simulink model "power_shuffler_sim"  (R2025b)
settings: Solver=VariableStepAuto  StartTime=0.0  StopTime=0.15  MaxStep=1e-4  RelTol=1e-4
PreLoadFcn:
  | P = init_params; CTRL_MODE = 1;
libraries: fl_lib x74, ee_lib x53, nesl_utility x50
(part 1 of 6)
settings Model: SimulationMode=accelerator  Creator=jazsa  LastModifiedBy=jazsa
settings SolverCC: ZeroCrossAlgorithm=Adaptive
settings DataIOCC: SignalLogging=off

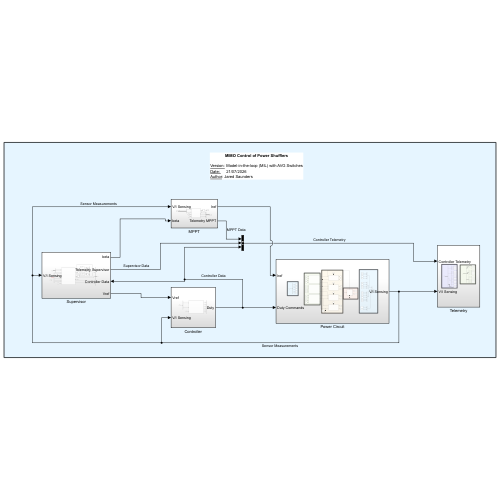
[thumbnail: Simulink's stored preview of the top-level diagram]
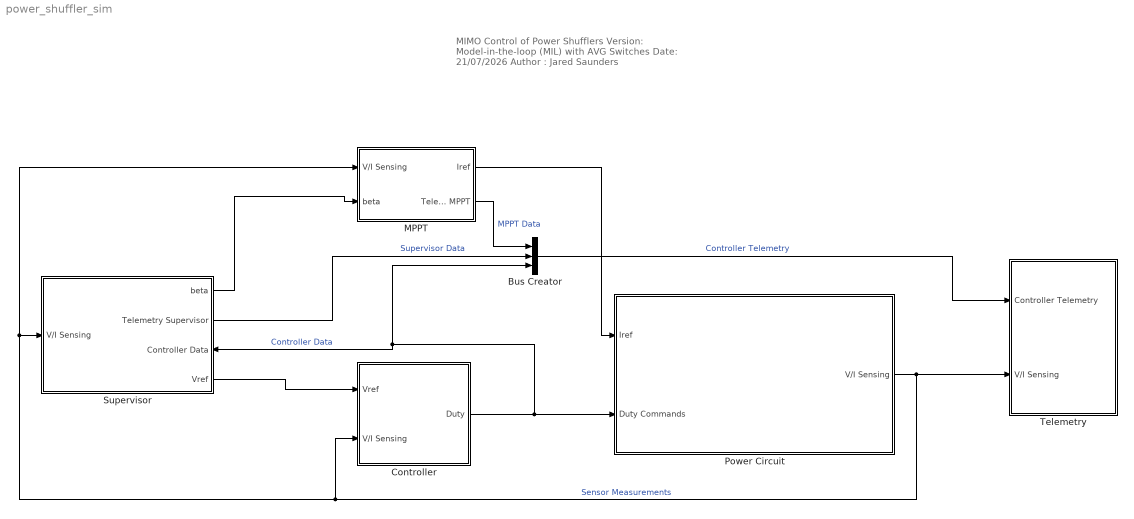
== system power_shuffler_sim ==
  note: MIMO Control of Power Shufflers
      |
      | Version: Model-in-the-loop (MIL) with AVG Switches
      | Date: 21/07/2026
      | Author : Jared Saunders
  Bus Creator : BusCreator  Inputs=3
  Controller : Subsystem
  MPPT : Subsystem
  Power Circuit : Subsystem
  Supervisor : Subsystem
      settings: PortSchema="{\"entries\":[{\"content\":{\"sides\":[{\"content\":{\"connectorIds\":[\"In1\"]},\"type\":\"ConnectorPlacement.EquallySpacedRectSide\",\"uuid\":\"4149ece3-2139-4a6b-be3b-85e3b5016338\"},{\"content\":{\"connectorIds\":[\"Out1\",\"Out2\",\"In2\",\"Out3\"],\"side\":\"RIGHT\"},\"type\":\"ConnectorPlacement.EquallySpacedRectSide\",\"uuid\":\"a4c8f16e-63c5-4e73-b921-9be0544bd052\"},{\"content\":{\"side\":\"TOP\"},\"type\":\"ConnectorPlacement.EquallySpacedRectSide\",\"uuid\":\"efcb0ad6-b028-42ed-a2aa-71b179d48e39\"}]},\"type\":\"ConnectorPlacement.EquallySpacedConnector\",\"uuid\":\"3400d1fe-81e3-4212-a4bc-db484173b6e0\"}],\"packageUris\":[\"http://schema.mathworks.com/mf0/Connector/R2020b\"],\"version\":\"1.0\"}"
  Telemetry : Subsystem
  wires:
  MPPT/1(Iref) -> Power Circuit/1(Iref)
  Supervisor/1(beta) -> MPPT/2(beta)
  Power Circuit/1(V/I Sensing) -> Telemetry/2(V/I Sensing), Controller/2(V/I Sensing), MPPT/1(V/I Sensing), Supervisor/1(V/I Sensing)  "Sensor Measurements"
  Supervisor/3(Vref) -> Controller/1(Vref)
  Controller/1(Duty) -> Power Circuit/2(Duty Commands), Bus Creator/3, Supervisor/2(Controller Data)  "Controller Data"
  MPPT/2(Telemetry MPPT) -> Bus Creator/1  "MPPT Data"
  Supervisor/2(Telemetry Supervisor) -> Bus Creator/2  "Supervisor Data"
  Bus Creator/1 -> Telemetry/1(Controller Telemetry)  "Controller Telemetry"

== system power_shuffler_sim/Controller ==
  Vref : Inport
  V/I Sensing : Inport  Port=2
  Bus Creator : BusCreator  Inputs=6
  Bus Selector : BusSelector  OutputSignals=Module Voltages,Phase Currents
  Controller : MATLAB Function  TreatAsAtomicUnit=on  SystemSampleTime=50e-6
  Duty : Outport
  wires:
  Bus Selector/1 -> Controller/1(VM)  "<Module Voltages>"
  Controller/6(dB3) -> Bus Creator/6
  Controller/5(dA3) -> Bus Creator/5
  Controller/4(dB2) -> Bus Creator/4
  Controller/3(dA2) -> Bus Creator/3
  Controller/2(dB1) -> Bus Creator/2
  Controller/1(dA1) -> Bus Creator/1
  Bus Creator/1 -> Duty/1
  V/I Sensing/1 -> Bus Selector/1
  Bus Selector/2 -> Controller/2(IL)  "<Phase Currents>"
  Vref/1 -> Controller/3(rv)

== system power_shuffler_sim/MPPT ==
  V/I Sensing : Inport
  beta : Inport  Port=2
  Bus Creator : BusCreator  Inputs=3
  Bus Selector : BusSelector  OutputSignals=String Power Meter
  Bus Selector1 : BusSelector  OutputSignals=V_string,I_string
  Delay : UnitDelay  InitialCondition=12  SampleTime=1e-3  HasFrameUpgradeWarning=on
  Enable : Constant
  P&O : MATLAB Function  TreatAsAtomicUnit=on  SystemSampleTime=1e-3
  Iref : Outport
  Telemetry MPPT : Outport  Port=2
  wires:
  beta/1 -> P&O/3(beta)
  V/I Sensing/1 -> Bus Selector/1
  P&O/3(state) -> Bus Creator/3
  Bus Selector1/1 -> P&O/1(Vstr)  "<V_string>"
  Bus Selector1/2 -> P&O/2(Istr)  "<I_string>"
  P&O/1(Iref) -> Bus Creator/1, Delay/1
  Delay/1 -> Iref/1
  Enable/1 -> P&O/4(en)
  Bus Creator/1 -> Telemetry MPPT/1
  P&O/2(Pav) -> Bus Creator/2
  Bus Selector/1 -> Bus Selector1/1  "<String Power Meter>"

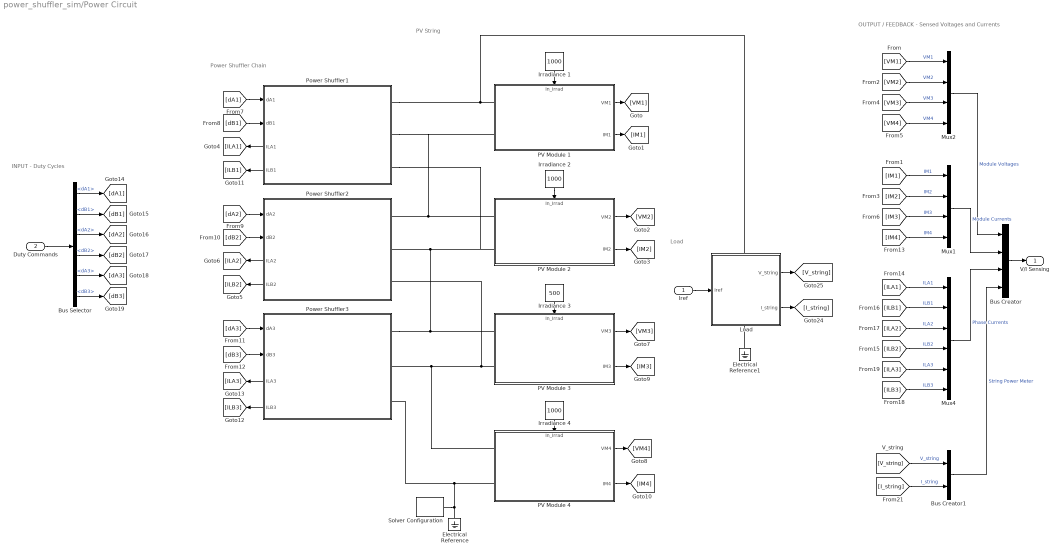
== system power_shuffler_sim/Power Circuit ==
  note: OUTPUT / FEEDBACK - Sensed Voltages and Currents
  note: Load
  note: PV String
  note: Power Shuffler Chain
  note: INPUT - Duty Cycles
  Iref : Inport
  Duty Commands : Inport  Port=2
  Bus Creator : BusCreator  Inputs=4
  Bus Creator1 : BusCreator  Inputs=2
  Bus Selector : BusSelector  OutputSignals=dA1,dB1,dA2,dB2,dA3,dB3
  Electrical Reference : fl_lib/Electrical/Electrical Elements/Electrical Reference
  Electrical Reference1 : fl_lib/Electrical/Electrical Elements/Electrical Reference
  Irradiance 1 : Constant  Value=1000
  Irradiance 2 : Constant  Value=1000
  Irradiance 3 : Constant  Value=500
  Irradiance 4 : Constant  Value=1000
  Load : Subsystem
      settings: PortSchema="{\"entries\":[{\"content\":{\"sides\":[{\"content\":{\"connectorIds\":[\"LConn1\"]},\"type\":\"ConnectorPlacement.EquallySpacedRectSide\",\"uuid\":\"6f5f716f-38b7-43f9-a9ba-568c6ccf5920\"},{\"content\":{\"connectorIds\":[\"RConn1\"],\"side\":\"RIGHT\"},\"type\":\"ConnectorPlacement.EquallySpacedRectSide\",\"uuid\":\"74a237b1-90a9-413f-978d-7052f4ba1489\"},{\"content\":{\"connectorIds\":[\"In1\"],\"side\":\"TOP\"},\"type\":\"ConnectorPlacement.EquallySpacedRectSide\",\"uuid\":\"e5fcb88f-496e-42e0-91fa-e640406c50d5\"},{\"content\":{\"connectorIds\":[\"Out1\",\"Out2\"],\"side\":\"BOTTOM\"},\"type\":\"ConnectorPlacement.EquallySpacedRectSide\",\"uuid\":\"aed6b45d-7ab9-4ae0-b4e0-d20dd58bb9bf\"}]},\"type\":\"ConnectorPlacement.EquallySpacedConnector\",\"uuid\":\"f6ffe9ce-5007-4054-8c52-fa2588b4e46b\"}],\"packageUris\":[\"http://schema.mathworks.com/mf0/Connector/R2020b\"],\"version\":\"1.0\"}"
  Mux1 : Mux
  Mux2 : Mux
  Mux4 : Mux  Inputs=6
  PV Module 1 : Subsystem
      settings: PortSchema="{\"entries\":[{\"content\":{\"sides\":[{\"content\":{\"connectorIds\":[\"LConn1\",\"LConn2\"]},\"type\":\"ConnectorPlacement.EquallySpacedRectSide\",\"uuid\":\"00bc81be-eb87-4e0d-8cf1-aaf392b111b3\"},{\"content\":{\"connectorIds\":[\"Out1\",\"Out2\"],\"side\":\"RIGHT\"},\"type\":\"ConnectorPlacement.EquallySpacedRectSide\",\"uuid\":\"136cfb59-61d1-4be5-a5a1-62fe670dfe2d\"},{\"content\":{\"connectorIds\":[\"In1\"],\"side\":\"TOP\"},\"type\":\"ConnectorPlacement.EquallySpacedRectSide\",\"uuid\":\"1fa490a3-fddf-446b-98a1-153f2ac018d8\"}]},\"type\":\"ConnectorPlacement.EquallySpacedConnector\",\"uuid\":\"e6ea07bf-3162-47e8-af67-1b2f68d57f24\"}],\"packageUris\":[\"http://schema.mathworks.com/mf0/Connector/R2020b\"],\"version\":\"1.0\"}"
  PV Module 2 : Subsystem
      settings: PortSchema="{\"entries\":[{\"content\":{\"sides\":[{\"content\":{\"connectorIds\":[\"LConn1\",\"LConn2\"]},\"type\":\"ConnectorPlacement.EquallySpacedRectSide\",\"uuid\":\"00bc81be-eb87-4e0d-8cf1-aaf392b111b3\"},{\"content\":{\"connectorIds\":[\"Out1\",\"Out2\"],\"side\":\"RIGHT\"},\"type\":\"ConnectorPlacement.EquallySpacedRectSide\",\"uuid\":\"136cfb59-61d1-4be5-a5a1-62fe670dfe2d\"},{\"content\":{\"connectorIds\":[\"In1\"],\"side\":\"TOP\"},\"type\":\"ConnectorPlacement.EquallySpacedRectSide\",\"uuid\":\"1fa490a3-fddf-446b-98a1-153f2ac018d8\"}]},\"type\":\"ConnectorPlacement.EquallySpacedConnector\",\"uuid\":\"e6ea07bf-3162-47e8-af67-1b2f68d57f24\"}],\"packageUris\":[\"http://schema.mathworks.com/mf0/Connector/R2020b\"],\"version\":\"1.0\"}"
  PV Module 3 : Subsystem
      settings: PortSchema="{\"entries\":[{\"content\":{\"sides\":[{\"content\":{\"connectorIds\":[\"LConn1\",\"LConn2\"]},\"type\":\"ConnectorPlacement.EquallySpacedRectSide\",\"uuid\":\"00bc81be-eb87-4e0d-8cf1-aaf392b111b3\"},{\"content\":{\"connectorIds\":[\"Out1\",\"Out2\"],\"side\":\"RIGHT\"},\"type\":\"ConnectorPlacement.EquallySpacedRectSide\",\"uuid\":\"136cfb59-61d1-4be5-a5a1-62fe670dfe2d\"},{\"content\":{\"connectorIds\":[\"In1\"],\"side\":\"TOP\"},\"type\":\"ConnectorPlacement.EquallySpacedRectSide\",\"uuid\":\"1fa490a3-fddf-446b-98a1-153f2ac018d8\"}]},\"type\":\"ConnectorPlacement.EquallySpacedConnector\",\"uuid\":\"e6ea07bf-3162-47e8-af67-1b2f68d57f24\"}],\"packageUris\":[\"http://schema.mathworks.com/mf0/Connector/R2020b\"],\"version\":\"1.0\"}"
  PV Module 4 : Subsystem
      settings: PortSchema="{\"entries\":[{\"content\":{\"sides\":[{\"content\":{\"connectorIds\":[\"LConn1\",\"LConn2\"]},\"type\":\"ConnectorPlacement.EquallySpacedRectSide\",\"uuid\":\"00bc81be-eb87-4e0d-8cf1-aaf392b111b3\"},{\"content\":{\"connectorIds\":[\"Out1\",\"Out2\"],\"side\":\"RIGHT\"},\"type\":\"ConnectorPlacement.EquallySpacedRectSide\",\"uuid\":\"136cfb59-61d1-4be5-a5a1-62fe670dfe2d\"},{\"content\":{\"connectorIds\":[\"In1\"],\"side\":\"TOP\"},\"type\":\"ConnectorPlacement.EquallySpacedRectSide\",\"uuid\":\"1fa490a3-fddf-446b-98a1-153f2ac018d8\"}]},\"type\":\"ConnectorPlacement.EquallySpacedConnector\",\"uuid\":\"e6ea07bf-3162-47e8-af67-1b2f68d57f24\"}],\"packageUris\":[\"http://schema.mathworks.com/mf0/Connector/R2020b\"],\"version\":\"1.0\"}"
  Power Shuffler1 : Subsystem
      settings: PortSchema="{\"entries\":[{\"content\":{\"sides\":[{\"content\":{\"connectorIds\":[\"LConn1\",\"LConn2\",\"LConn3\"]},\"type\":\"ConnectorPlacement.EquallySpacedRectSide\",\"uuid\":\"00177d11-8382-42fd-b27c-fc09158175e4\"},{\"content\":{\"connectorIds\":[\"In1\",\"In2\",\"Out1\",\"Out2\"],\"side\":\"RIGHT\"},\"type\":\"ConnectorPlacement.EquallySpacedRectSide\",\"uuid\":\"90a306f0-da10-41e1-a725-cfb753adc00c\"},{\"content\":{\"side\":\"TOP\"},\"type\":\"ConnectorPlacement.EquallySpacedRectSide\",\"uuid\":\"612e5683-3ee7-4398-9a5a-0cbdc6c6e41b\"}]},\"type\":\"ConnectorPlacement.EquallySpacedConnector\",\"uuid\":\"1790a0ac-9047-4198-9955-1e7cd181ed81\"}],\"packageUris\":[\"http://schema.mathworks.com/mf0/Connector/R2020b\"],\"version\":\"1.0\"}"
  Power Shuffler2 : Subsystem
      settings: PortSchema="{\"entries\":[{\"content\":{\"sides\":[{\"content\":{\"connectorIds\":[\"LConn1\",\"LConn2\",\"LConn3\"]},\"type\":\"ConnectorPlacement.EquallySpacedRectSide\",\"uuid\":\"00177d11-8382-42fd-b27c-fc09158175e4\"},{\"content\":{\"connectorIds\":[\"In1\",\"In2\",\"Out1\",\"Out2\"],\"side\":\"RIGHT\"},\"type\":\"ConnectorPlacement.EquallySpacedRectSide\",\"uuid\":\"90a306f0-da10-41e1-a725-cfb753adc00c\"},{\"content\":{\"side\":\"TOP\"},\"type\":\"ConnectorPlacement.EquallySpacedRectSide\",\"uuid\":\"612e5683-3ee7-4398-9a5a-0cbdc6c6e41b\"}]},\"type\":\"ConnectorPlacement.EquallySpacedConnector\",\"uuid\":\"1790a0ac-9047-4198-9955-1e7cd181ed81\"}],\"packageUris\":[\"http://schema.mathworks.com/mf0/Connector/R2020b\"],\"version\":\"1.0\"}"
  Power Shuffler3 : Subsystem
      settings: PortSchema="{\"entries\":[{\"content\":{\"sides\":[{\"content\":{\"connectorIds\":[\"LConn1\",\"LConn2\",\"LConn3\"]},\"type\":\"ConnectorPlacement.EquallySpacedRectSide\",\"uuid\":\"00177d11-8382-42fd-b27c-fc09158175e4\"},{\"content\":{\"connectorIds\":[\"In1\",\"In2\",\"Out1\",\"Out2\"],\"side\":\"RIGHT\"},\"type\":\"ConnectorPlacement.EquallySpacedRectSide\",\"uuid\":\"90a306f0-da10-41e1-a725-cfb753adc00c\"},{\"content\":{\"side\":\"TOP\"},\"type\":\"ConnectorPlacement.EquallySpacedRectSide\",\"uuid\":\"612e5683-3ee7-4398-9a5a-0cbdc6c6e41b\"}]},\"type\":\"ConnectorPlacement.EquallySpacedConnector\",\"uuid\":\"1790a0ac-9047-4198-9955-1e7cd181ed81\"}],\"packageUris\":[\"http://schema.mathworks.com/mf0/Connector/R2020b\"],\"version\":\"1.0\"}"
  Solver Configuration : nesl_utility/Solver Configuration  PhysicalDomain=network_engine_domain  SubClassName=solver  LeftPortType=input  RightPortType=generic  Tones=[]  Harmonics=[]  SimulateNoise=off  Profile=off  UseLocalSampling=off  EnableSwitchedLinearOptims=on  FrequencyDomain=off  UseCCode=off  RelTol=0.001  AbsTol=0.001  MinStep=1e-09  ToWorkspace=off  RevertToSquareIcSolve=off  NumHomotopyIterations=100  PhasorMode=off  PhasorModeNumHarmonics=1  ConsistencySolver=NEWTON_XTOL_AFTER_FTOL  IndexReductionMethod=DerivativeReplacement  DoDC=off  ResidualTolerance=1e-09  ConsistencyTolSource=GLOBAL  ConsistencyAbsTol=0.001  ConsistencyRelTol=0.001  ConsistencyTolFactor=0.001  UseLocalSolver=on  LocalSolverChoice=NE_BACKWARD_EULER_ADVANCER  ResolveIndetEquations=on  FunctionEvalNumThread=1  LocalSolverSampleTime=1e-7  DoFixedCost=off  MaxNonlinIter=3  MaxModeIter=2  ComputeImpulses=off  ImpulseIterations=2  LinearAlgebra=auto  LinearAlgebraNumThread=0  EquationFormulation=NE_TIME_EF  DelaysMemoryBudget=1024  AutomaticFiltering=on  FilteringTimeConstant=0.001  PartitionStorageMethod=AS_NEEDED  PartitionMemoryBudget=1024  PartitionMethod=ROBUST  MultibodyUseLocalSolver=off  MultibodyLocalSolverChoice=ODE1  MultibodyLocalSolverSampleTime=0.001
  V/I Sensing : Outport
  wires:
  Iref/1 -> Load/1(Iref)
  Load/2(V_String) -> [V_string]
  PV Module 1/1(VM1) -> [VM1]
  Load/1(I_string) -> [I_string]
  Irradiance 3/1 -> PV Module 3/1(In_Irrad)
  Irradiance 4/1 -> PV Module 4/1(In_Irrad)
  Irradiance 2/1 -> PV Module 2/1(In_Irrad)
  Irradiance 1/1 -> PV Module 1/1(In_Irrad)
  Mux2/1 -> Bus Creator/1  "Module Voltages"
  Mux1/1 -> Bus Creator/2  "Module Currents"
  [VM1] -> Mux2/1  "VM1"
  PV Module 1/2(IM1) -> [IM1]
  [IM1] -> Mux1/1  "IM1"
  PV Module 2/1(VM2) -> [VM2]
  [VM2] -> Mux2/2  "VM2"
  PV Module 2/2(IM2) -> [IM2]
  [VM3] -> Mux2/3  "VM3"
  [IM2] -> Mux1/2  "IM2"
  PV Module 3/1(VM3) -> [VM3]
  PV Module 4/1(VM4) -> [VM4]
  [VM4] -> Mux2/4  "VM4"
  PV Module 3/2(IM3) -> [IM3]
  [IM3] -> Mux1/3  "IM3"
  PV Module 4/2(IM4) -> [IM4]
  [IM4] -> Mux1/4  "IM4"
  Power Shuffler1/1(ILA1) -> [ILA1]
  Power Shuffler1/2(ILB1) -> [ILB1]
  Power Shuffler2/2(ILB2) -> [ILB2]
  Power Shuffler2/1(ILA2) -> [ILA2]
  Power Shuffler3/2(ILB3) -> [ILB3]
  Power Shuffler3/1(ILA3) -> [ILA3]
  [ILB3] -> Mux4/6  "ILB3"
  [ILA3] -> Mux4/5  "ILA3"
  [ILA1] -> Mux4/1  "ILA1"
  [ILA2] -> Mux4/3  "ILA2"
  [ILB1] -> Mux4/2  "ILB1"
  [ILB2] -> Mux4/4  "ILB2"
  Mux4/1 -> Bus Creator/3  "Phase Currents"
  [dA1] -> Power Shuffler1/1(dA1)
  Duty Commands/1 -> Bus Selector/1
  Bus Selector/1 -> [dA1]  "<dA1>"
  Bus Selector/2 -> [dB1]  "<dB1>"
  [dB1] -> Power Shuffler1/2(dB1)
  [dB2] -> Power Shuffler2/2(dB2)
  [dA2] -> Power Shuffler2/1(dA2)
  [dA3] -> Power Shuffler3/1(dA3)
  [dB3] -> Power Shuffler3/2(dB3)
  Bus Selector/4 -> [dB2]  "<dB2>"
  Bus Selector/3 -> [dA2]  "<dA2>"
  Bus Selector/6 -> [dB3]  "<dB3>"
  Bus Selector/5 -> [dA3]  "<dA3>"
  [V_string] -> Bus Creator1/1  "V_string"
  [I_string] -> Bus Creator1/2  "I_string"
  Bus Creator/1 -> V/I Sensing/1
  Bus Creator1/1 -> Bus Creator/4  "String Power Meter"
  connections:
  PV Module 1/LConn2 -- Power Shuffler1/LConn2 -- PV Module 2/LConn1 -- Power Shuffler2/LConn1
  PV Module 1/LConn1 -- Load/RConn1 -- Power Shuffler1/LConn1
  PV Module 3/LConn1 -- PV Module 2/LConn2 -- Power Shuffler1/LConn3 -- Power Shuffler2/LConn2 -- Power Shuffler3/LConn1
  Solver Configuration/RConn1 -- Power Shuffler3/LConn3 -- PV Module 4/LConn2 -- Electrical Reference/LConn1
  PV Module 3/LConn2 -- PV Module 4/LConn1 -- Power Shuffler3/LConn2 -- Power Shuffler2/LConn3
  Electrical Reference1/LConn1 -- Load/LConn1

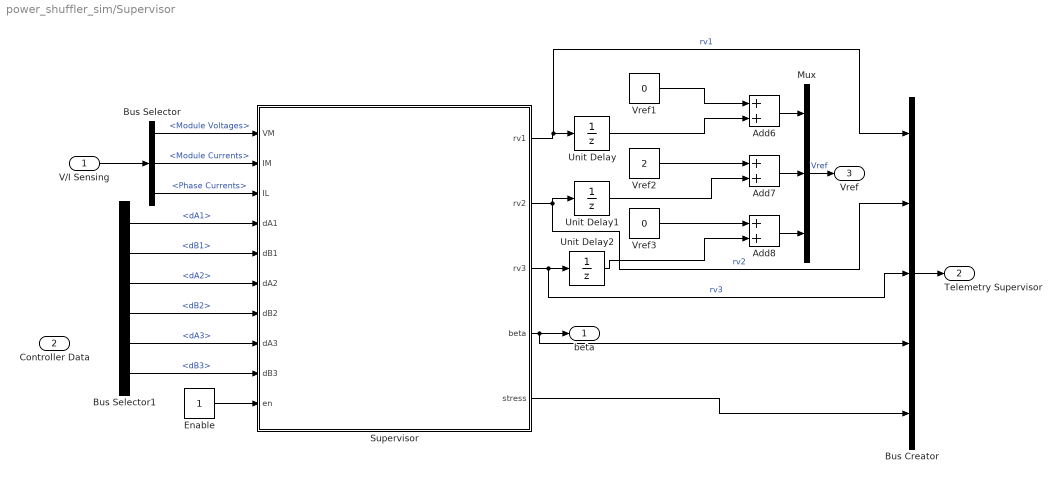
== system power_shuffler_sim/Supervisor ==
  V/I Sensing : Inport
  Controller Data : Inport  Port=2
  Add6 : Sum
  Add7 : Sum
  Add8 : Sum
  Bus Creator : BusCreator  Inputs=5
  Bus Selector : BusSelector  OutputSignals=Module Voltages,Module Currents,Phase Currents
  Bus Selector1 : BusSelector  OutputSignals=dA1,dB1,dA2,dB2,dA3,dB3
  Enable : Constant
  Mux : Mux  Inputs=3
  Supervisor : MATLAB Function  TreatAsAtomicUnit=on  SystemSampleTime=1e-3
  Unit Delay : UnitDelay  SampleTime=1e-3  HasFrameUpgradeWarning=on
  Unit Delay1 : UnitDelay  SampleTime=1e-3  HasFrameUpgradeWarning=on
  Unit Delay2 : UnitDelay  SampleTime=1e-3  HasFrameUpgradeWarning=on
  Vref1 : Constant  Value=0
  Vref2 : Constant  Value=2
  Vref3 : Constant  Value=0
  beta : Outport
  Telemetry Supervisor : Outport  Port=2
  Vref : Outport  Port=3
  wires:
  Bus Selector/3 -> Supervisor/3(IL)  "<Phase Currents>"
  Bus Creator/1 -> Telemetry Supervisor/1
  Bus Selector1/4 -> Supervisor/7(dB2)  "<dB2>"
  ? -> Bus Selector1/1
  Bus Selector1/5 -> Supervisor/8(dA3)  "<dA3>"
  Bus Selector1/6 -> Supervisor/9(dB3)  "<dB3>"
  Add6/1 -> Mux/1
  Bus Selector/2 -> Supervisor/2(IM)  "<Module Currents>"
  Add8/1 -> Mux/3
  Vref1/1 -> Add6/1
  Vref2/1 -> Add7/1
  Add7/1 -> Mux/2
  V/I Sensing/1 -> Bus Selector/1
  Enable/1 -> Supervisor/10(en)
  Supervisor/5(stress) -> Bus Creator/5
  Supervisor/2(rv2) -> Unit Delay1/1, Bus Creator/2  "rv2"
  Unit Delay1/1 -> Add7/2
  Bus Selector1/1 -> Supervisor/4(dA1)  "<dA1>"
  Bus Selector/1 -> Supervisor/1(VM)  "<Module Voltages>"
  Vref3/1 -> Add8/1
  Supervisor/1(rv1) -> Bus Creator/1, Unit Delay/1  "rv1"
  Unit Delay2/1 -> Add8/2
  Supervisor/4(beta) -> beta/1, Bus Creator/4
  Mux/1 -> Vref/1  "Vref"
  Bus Selector1/3 -> Supervisor/6(dA2)  "<dA2>"
  Unit Delay/1 -> Add6/2
  Supervisor/3(rv3) -> Bus Creator/3, Unit Delay2/1  "rv3"
  Bus Selector1/2 -> Supervisor/5(dB1)  "<dB1>"

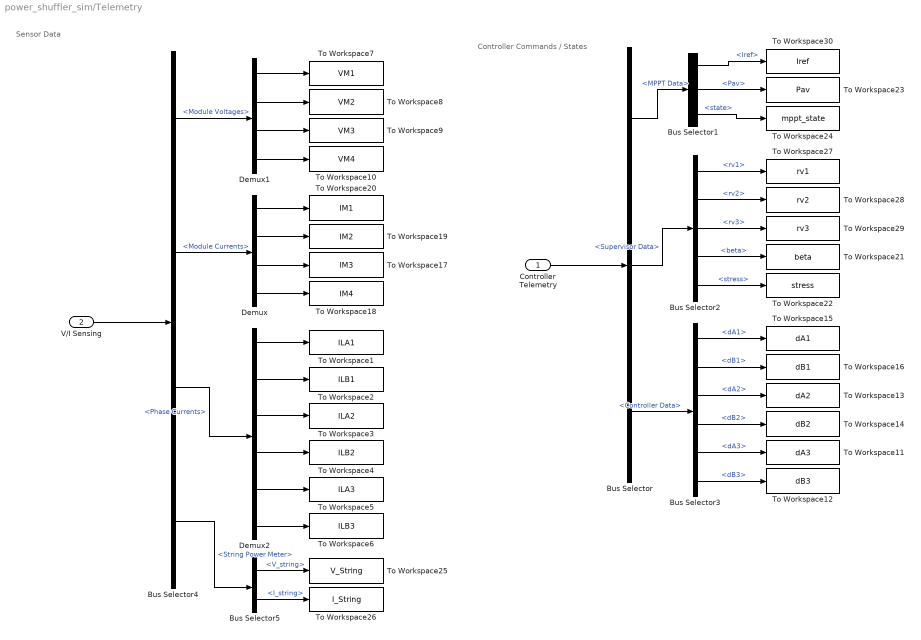
== system power_shuffler_sim/Telemetry ==
  note: Controller Commands / States
  note: Sensor Data
  Controller Telemetry : Inport
  V/I Sensing : Inport  Port=2
  Bus Selector : BusSelector  OutputSignals=MPPT Data,Supervisor Data,Controller Data
  Bus Selector1 : BusSelector  OutputSignals=Iref,Pav,state
  Bus Selector2 : BusSelector  OutputSignals=rv1,rv2,rv3,beta,stress
  Bus Selector3 : BusSelector  OutputSignals=dA1,dB1,dA2,dB2,dA3,dB3
  Bus Selector4 : BusSelector  OutputSignals=Module Voltages,Module Currents,Phase Currents,String Power Meter
  Bus Selector5 : BusSelector  OutputSignals=V_string,I_string
  Demux : Demux
  Demux1 : Demux
  Demux2 : Demux  Outputs=6
  To Workspace1 : ToWorkspace  VariableName=ILA1  SaveFormat=Timeseries  SampleTime=-1
  To Workspace10 : ToWorkspace  VariableName=VM4  SaveFormat=Timeseries  SampleTime=-1
  To Workspace11 : ToWorkspace  VariableName=dA3  SaveFormat=Timeseries  SampleTime=-1
  To Workspace12 : ToWorkspace  VariableName=dB3  SaveFormat=Timeseries  SampleTime=-1
  To Workspace13 : ToWorkspace  VariableName=dA2  SaveFormat=Timeseries  SampleTime=-1
  To Workspace14 : ToWorkspace  VariableName=dB2  SaveFormat=Timeseries  SampleTime=-1
  To Workspace15 : ToWorkspace  VariableName=dA1  SaveFormat=Timeseries  SampleTime=-1
  To Workspace16 : ToWorkspace  VariableName=dB1  SaveFormat=Timeseries  SampleTime=-1
  To Workspace17 : ToWorkspace  VariableName=IM3  SaveFormat=Timeseries  SampleTime=-1
  To Workspace18 : ToWorkspace  VariableName=IM4  SaveFormat=Timeseries  SampleTime=-1
  To Workspace19 : ToWorkspace  VariableName=IM2  SaveFormat=Timeseries  SampleTime=-1
  To Workspace2 : ToWorkspace  VariableName=ILB1  SaveFormat=Timeseries  SampleTime=-1
  To Workspace20 : ToWorkspace  VariableName=IM1  SaveFormat=Timeseries  SampleTime=-1
  To Workspace21 : ToWorkspace  VariableName=beta  SaveFormat=Timeseries  SampleTime=-1
  To Workspace22 : ToWorkspace  VariableName=stress  SaveFormat=Timeseries  SampleTime=-1
  To Workspace23 : ToWorkspace  VariableName=Pav  SaveFormat=Timeseries  SampleTime=-1
  To Workspace24 : ToWorkspace  VariableName=mppt_state  SaveFormat=Timeseries  SampleTime=-1
  To Workspace25 : ToWorkspace  VariableName=V_String  SaveFormat=Timeseries  SampleTime=-1
  To Workspace26 : ToWorkspace  VariableName=I_String  SaveFormat=Timeseries  SampleTime=-1
  To Workspace27 : ToWorkspace  VariableName=rv1  SaveFormat=Timeseries  SampleTime=-1
  To Workspace28 : ToWorkspace  VariableName=rv2  SaveFormat=Timeseries  SampleTime=-1
  To Workspace29 : ToWorkspace  VariableName=rv3  SaveFormat=Timeseries  SampleTime=-1
  To Workspace3 : ToWorkspace  VariableName=ILA2  SaveFormat=Timeseries  SampleTime=-1
  To Workspace30 : ToWorkspace  VariableName=Iref  SaveFormat=Timeseries  SampleTime=-1
  To Workspace4 : ToWorkspace  VariableName=ILB2  SaveFormat=Timeseries  SampleTime=-1
  To Workspace5 : ToWorkspace  VariableName=ILA3  SaveFormat=Timeseries  SampleTime=-1
  To Workspace6 : ToWorkspace  VariableName=ILB3  SaveFormat=Timeseries  SampleTime=-1
  To Workspace7 : ToWorkspace  VariableName=VM1  SaveFormat=Timeseries  SampleTime=-1
  To Workspace8 : ToWorkspace  VariableName=VM2  SaveFormat=Timeseries  SampleTime=-1
  To Workspace9 : ToWorkspace  VariableName=VM3  SaveFormat=Timeseries  SampleTime=-1
  wires:
  Bus Selector2/2 -> To Workspace28/1  "<rv2>"
  Bus Selector4/3 -> Demux2/1  "<Phase Currents>"
  Demux2/5 -> To Workspace5/1
  Demux/1 -> To Workspace20/1
  Demux1/2 -> To Workspace8/1
  Bus Selector/3 -> Bus Selector3/1  "<Controller Data>"
  Bus Selector3/1 -> To Workspace15/1  "<dA1>"
  Demux1/3 -> To Workspace9/1
  Bus Selector/1 -> Bus Selector1/1  "<MPPT Data>"
  Demux2/1 -> To Workspace1/1
  Bus Selector4/2 -> Demux/1  "<Module Currents>"
  Bus Selector5/2 -> To Workspace26/1  "<I_string>"
  Demux1/4 -> To Workspace10/1
  Bus Selector2/1 -> To Workspace27/1  "<rv1>"
  Demux2/3 -> To Workspace3/1
  Bus Selector3/6 -> To Workspace12/1  "<dB3>"
  Bus Selector2/4 -> To Workspace21/1  "<beta>"
  Demux2/2 -> To Workspace2/1
  Demux/3 -> To Workspace17/1
  Bus Selector3/3 -> To Workspace13/1  "<dA2>"
  Bus Selector2/3 -> To Workspace29/1  "<rv3>"
  Bus Selector3/2 -> To Workspace16/1  "<dB1>"
  Bus Selector5/1 -> To Workspace25/1  "<V_string>"
  Demux2/6 -> To Workspace6/1
  V/I Sensing/1 -> Bus Selector4/1
  Demux/4 -> To Workspace18/1
  Bus Selector4/4 -> Bus Selector5/1  "<String Power Meter>"
  Bus Selector3/5 -> To Workspace11/1  "<dA3>"
  Bus Selector/2 -> Bus Selector2/1  "<Supervisor Data>"
  Controller Telemetry/1 -> Bus Selector/1
  Demux2/4 -> To Workspace4/1
  Bus Selector1/2 -> To Workspace23/1  "<Pav>"
  Demux1/1 -> To Workspace7/1
  Bus Selector1/1 -> To Workspace30/1  "<Iref>"
  Bus Selector2/5 -> To Workspace22/1  "<stress>"
  Bus Selector3/4 -> To Workspace14/1  "<dB2>"
  Bus Selector1/3 -> To Workspace24/1  "<state>"
  Demux/2 -> To Workspace19/1
  Bus Selector4/1 -> Demux1/1  "<Module Voltages>"

== system power_shuffler_sim/Power Circuit/Load ==
  Iref : Inport
  Controlled Current Source : fl_lib/Electrical/Electrical Sources/Controlled Current Source
  Current Sensor : fl_lib/Electrical/Electrical Sensors/Current Sensor
  PS-Simulink Converter : nesl_utility/PS-Simulink Converter  PhysicalDomain=network_engine_domain  SubClassName=ps_output  LeftPortType=input  RightPortType=output  PseudoPeriodic=off  Frequencies=[]  VectorFormat=inherit  Unit=inherit  AffineConversion=off
  PS-Simulink Converter1 : nesl_utility/PS-Simulink Converter  PhysicalDomain=network_engine_domain  SubClassName=ps_output  LeftPortType=input  RightPortType=output  PseudoPeriodic=off  Frequencies=[]  VectorFormat=inherit  Unit=inherit  AffineConversion=off
  Simulink-PS Converter : nesl_utility/Simulink-PS Converter  PhysicalDomain=network_engine_domain  SubClassName=ps_input  LeftPortType=input  RightPortType=output  PseudoPeriodic=off  Frequencies=[]  NoiseDistribution=none  NoiseParameters=[]  Unit=1  AffineConversion=off  FilteringAndDerivatives=provide  SimscapeFilterOrder=1  InputFilterTimeConstant=0.001  UdotUserProvided=0
  Voltage Sensor : fl_lib/Electrical/Electrical Sensors/Voltage Sensor
  -ve Terminal : PMIOPort  Side=Left
  +Ve Terminal : PMIOPort  Port=2  Side=Right
  I_string : Outport
  V_String : Outport  Port=2
  wires:
  PS-Simulink Converter/1 -> V_String/1
  PS-Simulink Converter1/1 -> I_string/1
  Iref/1 -> Simulink-PS Converter/1
  connections:
  Voltage Sensor/RConn1 -- PS-Simulink Converter/LConn1
  +Ve Terminal/RConn1 -- Controlled Current Source/RConn2 -- Voltage Sensor/LConn1
  Voltage Sensor/RConn2 -- Current Sensor/RConn2 -- -ve Terminal/RConn1
  Current Sensor/RConn1 -- PS-Simulink Converter1/LConn1
  Controlled Current Source/LConn1 -- Current Sensor/LConn1
  Simulink-PS Converter/RConn1 -- Controlled Current Source/RConn1

== system power_shuffler_sim/Power Circuit/PV Module 1 ==
  In_Irrad : Inport
  Current Sensor : fl_lib/Electrical/Electrical Sensors/Current Sensor
  Diode : ee_lib/Semiconductors & Converters/Diode  ModelType=ee.enum.diode.modelType.pwl  TableType=ee.enum.diode.tableType.IfMat  IfMat=[.07, .12, .19, 1.75, 4.24, 7.32, 11.2; .16, .3, .72, 2.14, 5.02, 8.35, 13.12] A  VfMat=[.9, 1.15, 1.25, 1.5, 1.75, 2.17, 2.6, 2.85; .58, .68, .75, 1.1, 1.38, 1.77, 2.27, 2.7] V  TjVec=[25, 125] degC  VfVec=[.5, .7, .9, 1.3, 1.7, 2.1, 2.5] V  IfVec=[.1, .2, .5, 1, 2, 4, 7, 10] A  IrMat=[1e-06, 2e-06, 5e-06, 1e-05, 2.5e-05, 5e-05, .0001; 2e-06, 5e-06, 1e-05, 4e-05, 8e-05, .0002, .0005] A  VrMat=[10, 100, 200, 250, 300, 325, 350; 10, 70, 160, 220, 270, 300, 320] V  VrVec=[10, 20, 40, 50, 70, 80, 100] V  IrVec=[1e-06, 2e-06, 5e-06, 1e-05, 2e-05, 5e-05, .0001] A  Vf=0.6 V  Ron=0.3 Ohm  Goff=1e-8 S  prmExp=ee.enum.diode.expParam.useTwo  I12=[.0137, .545] A  V12=[.6, .7] V  RS=0 Ohm  Tmeas=298.15 K  IS=1e-12 A  ec=1  I1=0.0137 A  V1=0.6 V  N_series=1  N_parallel=1  ZenerEnable=false  Rz=0.3 Ohm  BV=inf V  C_param=ee.enum.diode.capParam.fixed  CJ=0 pF  CJ0=5 pF  Vvec=[.1, 10, 100] V  Cvec=[3.5, 1, .4] pF  VJ=1 V  Mgrad=0.5  FC=0.5  Q_param=ee.enum.diode.recoveryParam.off  iRM=-7.15 A  iF=4 A  didt=-750 A/us  trr_factor=3  trr=115 ns  Qrr=150 nA*s  Vr=-600 V  Ls=150 nH  Erec=0.03 J  TT=50 ns  tau=100 ns  T_param=ee.enum.diode.temperatureParam.off  Tdevice=298.15 K  I1_T2=0.245 A  V1_T2=0.5 V  IS_T2=1.25e-7 A  Tmeas2=125 degC  XTI_param=ee.enum.diode.xtiParam.pn  XTI=3  EG_param=ee.enum.diode.egapParam.material_si  EG=1.11 eV  dBVdT=0 V/K  enable_fault_input=simscape.enum.onoff.off  i_specify=off  i_priority=None  i=0 A  i_nominal_specify=off  i_nominal_value=1  i_nominal_unit=A  v_specify=off  v_priority=None  v=0 V  v_nominal_specify=off  v_nominal_value=1  v_nominal_unit=V  v_capacitor_specify=off  v_capacitor_priority=None  v_capacitor=0 V  v_capacitor_nominal_specify=off  v_capacitor_nominal_value=1  v_capacitor_nominal_unit=V  Qj_specify=off  Qj_priority=High  Qj=0 C  Qj_nominal_specify=off  Qj_nominal_value=1  Qj_nominal_unit=C  i_diode_specify=off  i_diode_priority=None  i_diode=0 A  i_diode_nominal_specify=off  i_diode_nominal_value=1  i_diode_nominal_unit=A  v_diode_specify=off  v_diode_priority=None  v_diode=0 V  v_diode_nominal_specify=off  v_diode_nominal_value=1  v_diode_nominal_unit=V  i_capacitor_specify=off  i_capacitor_priority=None  i_capacitor=0 A  i_capacitor_nominal_specify=off  i_capacitor_nominal_value=1  i_capacitor_nominal_unit=A  power_dissipated_specify=off  power_dissipated_priority=None  power_dissipated=0 W  power_dissipated_nominal_specify=off  power_dissipated_nominal_value=1  power_dissipated_nominal_unit=W  fidelity_level=ee.enum.diode.fidelity.includeChargeDyn  rec_loss_model=ee.enum.diode.reverseRecoveryModel.fixed  ErecVal=0 J  scaleWithIandV=true  ErecMat=zeros(2, 3) J  TjrecVec=[298.15, 398.15] K  IfrecVec=[.1, 1, 10] A  IrecVal=10 A  VrecVal=10 V  tFilter=1 / 1000 / 100 s  thermal_network_parameterization=ee.enum.thermalNetworkTopology.junctionCase  Rth=[0, 10] K/W  Rth_Cauer=[1, 3, 10] K/W  Rth_Foster=[.08, .14, .22, .16] K/W  thermal_mass_parameterization=ee.enum.thermalNetwork.timeconstant  thermal_mass=[0, 1] J/K  thermal_mass_Cauer=[.1, .3, 1] J/K  thermal_mass_Foster=[.001, .005, .05, .5] J/K  thermal_time_constant=[0, 10] s  thermal_time_constant_Cauer=[1, 3, 10] s  thermal_time_constant_Foster=[7e-05, .0007, .01, .08] s  thermal_mass_initial_temperatures=[25, 25] degC  thermal_mass_initial_temperatures_Cauer=[25, 25, 25] degC  junction_thermal_mass=0.01 J/K  Tvec_initial_Foster=[25, 25, 25, 25] degC  no_thermal_network=0  junction_temperature_specify=off  junction_temperature_priority=None  junction_temperature=25 degC  junction_temperature_nominal_specify=off  junction_temperature_nominal_value=1  junction_temperature_nominal_unit=degC
  LPF Voltage: 2nd Order 20kHz : TransferFcn  Numerator=[(2*pi*20000)^2]  Denominator=[1, sqrt(2)*(2*pi*20000), (2*pi*20000)^2]
  PS-Simulink Converter : nesl_utility/PS-Simulink Converter  PhysicalDomain=network_engine_domain  SubClassName=ps_output  LeftPortType=input  RightPortType=output  PseudoPeriodic=off  Frequencies=[]  VectorFormat=inherit  Unit=inherit  AffineConversion=off
  PS-Simulink Converter1 : nesl_utility/PS-Simulink Converter  PhysicalDomain=network_engine_domain  SubClassName=ps_output  LeftPortType=input  RightPortType=output  PseudoPeriodic=off  Frequencies=[]  VectorFormat=inherit  Unit=inherit  AffineConversion=off
  Simulink-PS Converter : nesl_utility/Simulink-PS Converter  PhysicalDomain=network_engine_domain  SubClassName=ps_input  LeftPortType=input  RightPortType=output  PseudoPeriodic=off  Frequencies=[]  NoiseDistribution=none  NoiseParameters=[]  Unit=1  AffineConversion=off  FilteringAndDerivatives=provide  SimscapeFilterOrder=1  InputFilterTimeConstant=0.001  UdotUserProvided=0
  Solar Cell : ee_lib/Sources/Solar Cell  prm=ee.enum.sources.solar_cell_prm.fiveParameter  Isc=7.34 A  Voc=0.6 V  Is=1.728e-12 A  Is2=0 A  Iph=14.96 A  Ir0=1000 W/m^2  ec=1  N2=2  Rs=0.00263 Ohm  Rp=inf Ohm  N_series=60  N_parallel=1  TIPH1=0.0005 1/K  EG=1.11 eV  TXIS1=3  TXIS2=3  TRS1=0  TRP1=0  Tmeas=25 degC  TFIXED=25 degC  thermal_mass=100 J/K  initial_temperature=25 degC
  Voltage Sensor : fl_lib/Electrical/Electrical Sensors/Voltage Sensor
  +ve Terminal : PMIOPort  Side=Left
  -ve Terminal : PMIOPort  Port=2  Side=Left
  VM1 : Outport
  IM1 : Outport  Port=2
  wires:
  PS-Simulink Converter/1 -> IM1/1
  In_Irrad/1 -> Simulink-PS Converter/1
  PS-Simulink Converter1/1 -> LPF Voltage: 2nd Order 20kHz/1
  LPF Voltage: 2nd Order 20kHz/1 -> VM1/1
  connections:
  -ve Terminal/RConn1 -- Diode/LConn1 -- Voltage Sensor/RConn2 -- Solar Cell/RConn1
  Solar Cell/LConn2 -- Diode/RConn1 -- Current Sensor/LConn1
  Simulink-PS Converter/RConn1 -- Solar Cell/LConn1
  Current Sensor/RConn1 -- PS-Simulink Converter/LConn1
  Current Sensor/RConn2 -- Voltage Sensor/LConn1 -- +ve Terminal/RConn1
  Voltage Sensor/RConn1 -- PS-Simulink Converter1/LConn1

== system power_shuffler_sim/Power Circuit/PV Module 2 ==
  In_Irrad : Inport
  Current Sensor : fl_lib/Electrical/Electrical Sensors/Current Sensor
  Diode : ee_lib/Semiconductors & Converters/Diode  ModelType=ee.enum.diode.modelType.pwl  TableType=ee.enum.diode.tableType.IfMat  IfMat=[.07, .12, .19, 1.75, 4.24, 7.32, 11.2; .16, .3, .72, 2.14, 5.02, 8.35, 13.12] A  VfMat=[.9, 1.15, 1.25, 1.5, 1.75, 2.17, 2.6, 2.85; .58, .68, .75, 1.1, 1.38, 1.77, 2.27, 2.7] V  TjVec=[25, 125] degC  VfVec=[.5, .7, .9, 1.3, 1.7, 2.1, 2.5] V  IfVec=[.1, .2, .5, 1, 2, 4, 7, 10] A  IrMat=[1e-06, 2e-06, 5e-06, 1e-05, 2.5e-05, 5e-05, .0001; 2e-06, 5e-06, 1e-05, 4e-05, 8e-05, .0002, .0005] A  VrMat=[10, 100, 200, 250, 300, 325, 350; 10, 70, 160, 220, 270, 300, 320] V  VrVec=[10, 20, 40, 50, 70, 80, 100] V  IrVec=[1e-06, 2e-06, 5e-06, 1e-05, 2e-05, 5e-05, .0001] A  Vf=0.6 V  Ron=0.3 Ohm  Goff=1e-8 S  prmExp=ee.enum.diode.expParam.useTwo  I12=[.0137, .545] A  V12=[.6, .7] V  RS=0 Ohm  Tmeas=298.15 K  IS=1e-12 A  ec=1  I1=0.0137 A  V1=0.6 V  N_series=1  N_parallel=1  ZenerEnable=false  Rz=0.3 Ohm  BV=inf V  C_param=ee.enum.diode.capParam.fixed  CJ=0 pF  CJ0=5 pF  Vvec=[.1, 10, 100] V  Cvec=[3.5, 1, .4] pF  VJ=1 V  Mgrad=0.5  FC=0.5  Q_param=ee.enum.diode.recoveryParam.off  iRM=-7.15 A  iF=4 A  didt=-750 A/us  trr_factor=3  trr=115 ns  Qrr=150 nA*s  Vr=-600 V  Ls=150 nH  Erec=0.03 J  TT=50 ns  tau=100 ns  T_param=ee.enum.diode.temperatureParam.off  Tdevice=298.15 K  I1_T2=0.245 A  V1_T2=0.5 V  IS_T2=1.25e-7 A  Tmeas2=125 degC  XTI_param=ee.enum.diode.xtiParam.pn  XTI=3  EG_param=ee.enum.diode.egapParam.material_si  EG=1.11 eV  dBVdT=0 V/K  enable_fault_input=simscape.enum.onoff.off  i_specify=off  i_priority=None  i=0 A  i_nominal_specify=off  i_nominal_value=1  i_nominal_unit=A  v_specify=off  v_priority=None  v=0 V  v_nominal_specify=off  v_nominal_value=1  v_nominal_unit=V  v_capacitor_specify=off  v_capacitor_priority=None  v_capacitor=0 V  v_capacitor_nominal_specify=off  v_capacitor_nominal_value=1  v_capacitor_nominal_unit=V  Qj_specify=off  Qj_priority=High  Qj=0 C  Qj_nominal_specify=off  Qj_nominal_value=1  Qj_nominal_unit=C  i_diode_specify=off  i_diode_priority=None  i_diode=0 A  i_diode_nominal_specify=off  i_diode_nominal_value=1  i_diode_nominal_unit=A  v_diode_specify=off  v_diode_priority=None  v_diode=0 V  v_diode_nominal_specify=off  v_diode_nominal_value=1  v_diode_nominal_unit=V  i_capacitor_specify=off  i_capacitor_priority=None  i_capacitor=0 A  i_capacitor_nominal_specify=off  i_capacitor_nominal_value=1  i_capacitor_nominal_unit=A  power_dissipated_specify=off  power_dissipated_priority=None  power_dissipated=0 W  power_dissipated_nominal_specify=off  power_dissipated_nominal_value=1  power_dissipated_nominal_unit=W  fidelity_level=ee.enum.diode.fidelity.includeChargeDyn  rec_loss_model=ee.enum.diode.reverseRecoveryModel.fixed  ErecVal=0 J  scaleWithIandV=true  ErecMat=zeros(2, 3) J  TjrecVec=[298.15, 398.15] K  IfrecVec=[.1, 1, 10] A  IrecVal=10 A  VrecVal=10 V  tFilter=1 / 1000 / 100 s  thermal_network_parameterization=ee.enum.thermalNetworkTopology.junctionCase  Rth=[0, 10] K/W  Rth_Cauer=[1, 3, 10] K/W  Rth_Foster=[.08, .14, .22, .16] K/W  thermal_mass_parameterization=ee.enum.thermalNetwork.timeconstant  thermal_mass=[0, 1] J/K  thermal_mass_Cauer=[.1, .3, 1] J/K  thermal_mass_Foster=[.001, .005, .05, .5] J/K  thermal_time_constant=[0, 10] s  thermal_time_constant_Cauer=[1, 3, 10] s  thermal_time_constant_Foster=[7e-05, .0007, .01, .08] s  thermal_mass_initial_temperatures=[25, 25] degC  thermal_mass_initial_temperatures_Cauer=[25, 25, 25] degC  junction_thermal_mass=0.01 J/K  Tvec_initial_Foster=[25, 25, 25, 25] degC  no_thermal_network=0  junction_temperature_specify=off  junction_temperature_priority=None  junction_temperature=25 degC  junction_temperature_nominal_specify=off  junction_temperature_nominal_value=1  junction_temperature_nominal_unit=degC
  LPF Voltage: 2nd Order 20kHz : TransferFcn  Numerator=[(2*pi*20000)^2]  Denominator=[1, sqrt(2)*(2*pi*20000), (2*pi*20000)^2]
  PS-Simulink Converter : nesl_utility/PS-Simulink Converter  PhysicalDomain=network_engine_domain  SubClassName=ps_output  LeftPortType=input  RightPortType=output  PseudoPeriodic=off  Frequencies=[]  VectorFormat=inherit  Unit=inherit  AffineConversion=off
  PS-Simulink Converter1 : nesl_utility/PS-Simulink Converter  PhysicalDomain=network_engine_domain  SubClassName=ps_output  LeftPortType=input  RightPortType=output  PseudoPeriodic=off  Frequencies=[]  VectorFormat=inherit  Unit=inherit  AffineConversion=off
  Simulink-PS Converter : nesl_utility/Simulink-PS Converter  PhysicalDomain=network_engine_domain  SubClassName=ps_input  LeftPortType=input  RightPortType=output  PseudoPeriodic=off  Frequencies=[]  NoiseDistribution=none  NoiseParameters=[]  Unit=1  AffineConversion=off  FilteringAndDerivatives=provide  SimscapeFilterOrder=1  InputFilterTimeConstant=0.001  UdotUserProvided=0
  Solar Cell : ee_lib/Sources/Solar Cell  prm=ee.enum.sources.solar_cell_prm.fiveParameter  Isc=7.34 A  Voc=0.6 V  Is=1.728e-12 A  Is2=0 A  Iph=14.96 A  Ir0=1000 W/m^2  ec=1  N2=2  Rs=0.00263 Ohm  Rp=inf Ohm  N_series=60  N_parallel=1  TIPH1=0.0005 1/K  EG=1.11 eV  TXIS1=3  TXIS2=3  TRS1=0  TRP1=0  Tmeas=25 degC  TFIXED=25 degC  thermal_mass=100 J/K  initial_temperature=25 degC
  Voltage Sensor : fl_lib/Electrical/Electrical Sensors/Voltage Sensor
  +ve Terminal : PMIOPort  Side=Left
  -ve Terminal : PMIOPort  Port=2  Side=Left
  VM2 : Outport
  IM2 : Outport  Port=2
  wires:
  In_Irrad/1 -> Simulink-PS Converter/1
  PS-Simulink Converter1/1 -> LPF Voltage: 2nd Order 20kHz/1
  PS-Simulink Converter/1 -> IM2/1
  LPF Voltage: 2nd Order 20kHz/1 -> VM2/1
  connections:
  -ve Terminal/RConn1 -- Diode/LConn1 -- Voltage Sensor/RConn2 -- Solar Cell/RConn1
  Solar Cell/LConn2 -- Diode/RConn1 -- Current Sensor/LConn1
  Simulink-PS Converter/RConn1 -- Solar Cell/LConn1
  Current Sensor/RConn2 -- Voltage Sensor/LConn1 -- +ve Terminal/RConn1
  Voltage Sensor/RConn1 -- PS-Simulink Converter1/LConn1
  PS-Simulink Converter/LConn1 -- Current Sensor/RConn1

== system power_shuffler_sim/Power Circuit/PV Module 3 ==
  In_Irrad : Inport
  Current Sensor : fl_lib/Electrical/Electrical Sensors/Current Sensor
  Diode : ee_lib/Semiconductors & Converters/Diode  ModelType=ee.enum.diode.modelType.pwl  TableType=ee.enum.diode.tableType.IfMat  IfMat=[.07, .12, .19, 1.75, 4.24, 7.32, 11.2; .16, .3, .72, 2.14, 5.02, 8.35, 13.12] A  VfMat=[.9, 1.15, 1.25, 1.5, 1.75, 2.17, 2.6, 2.85; .58, .68, .75, 1.1, 1.38, 1.77, 2.27, 2.7] V  TjVec=[25, 125] degC  VfVec=[.5, .7, .9, 1.3, 1.7, 2.1, 2.5] V  IfVec=[.1, .2, .5, 1, 2, 4, 7, 10] A  IrMat=[1e-06, 2e-06, 5e-06, 1e-05, 2.5e-05, 5e-05, .0001; 2e-06, 5e-06, 1e-05, 4e-05, 8e-05, .0002, .0005] A  VrMat=[10, 100, 200, 250, 300, 325, 350; 10, 70, 160, 220, 270, 300, 320] V  VrVec=[10, 20, 40, 50, 70, 80, 100] V  IrVec=[1e-06, 2e-06, 5e-06, 1e-05, 2e-05, 5e-05, .0001] A  Vf=0.6 V  Ron=0.3 Ohm  Goff=1e-8 S  prmExp=ee.enum.diode.expParam.useTwo  I12=[.0137, .545] A  V12=[.6, .7] V  RS=0 Ohm  Tmeas=298.15 K  IS=1e-12 A  ec=1  I1=0.0137 A  V1=0.6 V  N_series=1  N_parallel=1  ZenerEnable=false  Rz=0.3 Ohm  BV=inf V  C_param=ee.enum.diode.capParam.fixed  CJ=0 pF  CJ0=5 pF  Vvec=[.1, 10, 100] V  Cvec=[3.5, 1, .4] pF  VJ=1 V  Mgrad=0.5  FC=0.5  Q_param=ee.enum.diode.recoveryParam.off  iRM=-7.15 A  iF=4 A  didt=-750 A/us  trr_factor=3  trr=115 ns  Qrr=150 nA*s  Vr=-600 V  Ls=150 nH  Erec=0.03 J  TT=50 ns  tau=100 ns  T_param=ee.enum.diode.temperatureParam.off  Tdevice=298.15 K  I1_T2=0.245 A  V1_T2=0.5 V  IS_T2=1.25e-7 A  Tmeas2=125 degC  XTI_param=ee.enum.diode.xtiParam.pn  XTI=3  EG_param=ee.enum.diode.egapParam.material_si  EG=1.11 eV  dBVdT=0 V/K  enable_fault_input=simscape.enum.onoff.off  i_specify=off  i_priority=None  i=0 A  i_nominal_specify=off  i_nominal_value=1  i_nominal_unit=A  v_specify=off  v_priority=None  v=0 V  v_nominal_specify=off  v_nominal_value=1  v_nominal_unit=V  v_capacitor_specify=off  v_capacitor_priority=None  v_capacitor=0 V  v_capacitor_nominal_specify=off  v_capacitor_nominal_value=1  v_capacitor_nominal_unit=V  Qj_specify=off  Qj_priority=High  Qj=0 C  Qj_nominal_specify=off  Qj_nominal_value=1  Qj_nominal_unit=C  i_diode_specify=off  i_diode_priority=None  i_diode=0 A  i_diode_nominal_specify=off  i_diode_nominal_value=1  i_diode_nominal_unit=A  v_diode_specify=off  v_diode_priority=None  v_diode=0 V  v_diode_nominal_specify=off  v_diode_nominal_value=1  v_diode_nominal_unit=V  i_capacitor_specify=off  i_capacitor_priority=None  i_capacitor=0 A  i_capacitor_nominal_specify=off  i_capacitor_nominal_value=1  i_capacitor_nominal_unit=A  power_dissipated_specify=off  power_dissipated_priority=None  power_dissipated=0 W  power_dissipated_nominal_specify=off  power_dissipated_nominal_value=1  power_dissipated_nominal_unit=W  fidelity_level=ee.enum.diode.fidelity.includeChargeDyn  rec_loss_model=ee.enum.diode.reverseRecoveryModel.fixed  ErecVal=0 J  scaleWithIandV=true  ErecMat=zeros(2, 3) J  TjrecVec=[298.15, 398.15] K  IfrecVec=[.1, 1, 10] A  IrecVal=10 A  VrecVal=10 V  tFilter=1 / 1000 / 100 s  thermal_network_parameterization=ee.enum.thermalNetworkTopology.junctionCase  Rth=[0, 10] K/W  Rth_Cauer=[1, 3, 10] K/W  Rth_Foster=[.08, .14, .22, .16] K/W  thermal_mass_parameterization=ee.enum.thermalNetwork.timeconstant  thermal_mass=[0, 1] J/K  thermal_mass_Cauer=[.1, .3, 1] J/K  thermal_mass_Foster=[.001, .005, .05, .5] J/K  thermal_time_constant=[0, 10] s  thermal_time_constant_Cauer=[1, 3, 10] s  thermal_time_constant_Foster=[7e-05, .0007, .01, .08] s  thermal_mass_initial_temperatures=[25, 25] degC  thermal_mass_initial_temperatures_Cauer=[25, 25, 25] degC  junction_thermal_mass=0.01 J/K  Tvec_initial_Foster=[25, 25, 25, 25] degC  no_thermal_network=0  junction_temperature_specify=off  junction_temperature_priority=None  junction_temperature=25 degC  junction_temperature_nominal_specify=off  junction_temperature_nominal_value=1  junction_temperature_nominal_unit=degC
  LPF Voltage: 2nd Order 20kHz : TransferFcn  Numerator=[(2*pi*20000)^2]  Denominator=[1, sqrt(2)*(2*pi*20000), (2*pi*20000)^2]
  PS-Simulink Converter : nesl_utility/PS-Simulink Converter  PhysicalDomain=network_engine_domain  SubClassName=ps_output  LeftPortType=input  RightPortType=output  PseudoPeriodic=off  Frequencies=[]  VectorFormat=inherit  Unit=inherit  AffineConversion=off
  PS-Simulink Converter1 : nesl_utility/PS-Simulink Converter  PhysicalDomain=network_engine_domain  SubClassName=ps_output  LeftPortType=input  RightPortType=output  PseudoPeriodic=off  Frequencies=[]  VectorFormat=inherit  Unit=inherit  AffineConversion=off
  Simulink-PS Converter : nesl_utility/Simulink-PS Converter  PhysicalDomain=network_engine_domain  SubClassName=ps_input  LeftPortType=input  RightPortType=output  PseudoPeriodic=off  Frequencies=[]  NoiseDistribution=none  NoiseParameters=[]  Unit=1  AffineConversion=off  FilteringAndDerivatives=provide  SimscapeFilterOrder=1  InputFilterTimeConstant=0.001  UdotUserProvided=0
  Solar Cell : ee_lib/Sources/Solar Cell  prm=ee.enum.sources.solar_cell_prm.fiveParameter  Isc=7.34 A  Voc=0.6 V  Is=1.728e-12 A  Is2=0 A  Iph=14.96 A  Ir0=1000 W/m^2  ec=1  N2=2  Rs=0.00263 Ohm  Rp=inf Ohm  N_series=60  N_parallel=1  TIPH1=0.0005 1/K  EG=1.11 eV  TXIS1=3  TXIS2=3  TRS1=0  TRP1=0  Tmeas=25 degC  TFIXED=25 degC  thermal_mass=100 J/K  initial_temperature=25 degC
  Voltage Sensor : fl_lib/Electrical/Electrical Sensors/Voltage Sensor
  +ve Terminal : PMIOPort  Side=Left
  -ve Terminal : PMIOPort  Port=2  Side=Left
  VM3 : Outport
  IM3 : Outport  Port=2
  wires:
  PS-Simulink Converter/1 -> IM3/1
  In_Irrad/1 -> Simulink-PS Converter/1
  PS-Simulink Converter1/1 -> LPF Voltage: 2nd Order 20kHz/1
  LPF Voltage: 2nd Order 20kHz/1 -> VM3/1
  connections:
  -ve Terminal/RConn1 -- Diode/LConn1 -- Voltage Sensor/RConn2 -- Solar Cell/RConn1
  Solar Cell/LConn2 -- Diode/RConn1 -- Current Sensor/LConn1
  Simulink-PS Converter/RConn1 -- Solar Cell/LConn1
  Current Sensor/RConn1 -- PS-Simulink Converter/LConn1
  Current Sensor/RConn2 -- Voltage Sensor/LConn1 -- +ve Terminal/RConn1
  Voltage Sensor/RConn1 -- PS-Simulink Converter1/LConn1

== system power_shuffler_sim/Power Circuit/PV Module 4 ==
  In_Irrad : Inport
  Current Sensor : fl_lib/Electrical/Electrical Sensors/Current Sensor
  Diode : ee_lib/Semiconductors & Converters/Diode  ModelType=ee.enum.diode.modelType.pwl  TableType=ee.enum.diode.tableType.IfMat  IfMat=[.07, .12, .19, 1.75, 4.24, 7.32, 11.2; .16, .3, .72, 2.14, 5.02, 8.35, 13.12] A  VfMat=[.9, 1.15, 1.25, 1.5, 1.75, 2.17, 2.6, 2.85; .58, .68, .75, 1.1, 1.38, 1.77, 2.27, 2.7] V  TjVec=[25, 125] degC  VfVec=[.5, .7, .9, 1.3, 1.7, 2.1, 2.5] V  IfVec=[.1, .2, .5, 1, 2, 4, 7, 10] A  IrMat=[1e-06, 2e-06, 5e-06, 1e-05, 2.5e-05, 5e-05, .0001; 2e-06, 5e-06, 1e-05, 4e-05, 8e-05, .0002, .0005] A  VrMat=[10, 100, 200, 250, 300, 325, 350; 10, 70, 160, 220, 270, 300, 320] V  VrVec=[10, 20, 40, 50, 70, 80, 100] V  IrVec=[1e-06, 2e-06, 5e-06, 1e-05, 2e-05, 5e-05, .0001] A  Vf=0.6 V  Ron=0.3 Ohm  Goff=1e-8 S  prmExp=ee.enum.diode.expParam.useTwo  I12=[.0137, .545] A  V12=[.6, .7] V  RS=0 Ohm  Tmeas=298.15 K  IS=1e-12 A  ec=1  I1=0.0137 A  V1=0.6 V  N_series=1  N_parallel=1  ZenerEnable=false  Rz=0.3 Ohm  BV=inf V  C_param=ee.enum.diode.capParam.fixed  CJ=0 pF  CJ0=5 pF  Vvec=[.1, 10, 100] V  Cvec=[3.5, 1, .4] pF  VJ=1 V  Mgrad=0.5  FC=0.5  Q_param=ee.enum.diode.recoveryParam.off  iRM=-7.15 A  iF=4 A  didt=-750 A/us  trr_factor=3  trr=115 ns  Qrr=150 nA*s  Vr=-600 V  Ls=150 nH  Erec=0.03 J  TT=50 ns  tau=100 ns  T_param=ee.enum.diode.temperatureParam.off  Tdevice=298.15 K  I1_T2=0.245 A  V1_T2=0.5 V  IS_T2=1.25e-7 A  Tmeas2=125 degC  XTI_param=ee.enum.diode.xtiParam.pn  XTI=3  EG_param=ee.enum.diode.egapParam.material_si  EG=1.11 eV  dBVdT=0 V/K  enable_fault_input=simscape.enum.onoff.off  i_specify=off  i_priority=None  i=0 A  i_nominal_specify=off  i_nominal_value=1  i_nominal_unit=A  v_specify=off  v_priority=None  v=0 V  v_nominal_specify=off  v_nominal_value=1  v_nominal_unit=V  v_capacitor_specify=off  v_capacitor_priority=None  v_capacitor=0 V  v_capacitor_nominal_specify=off  v_capacitor_nominal_value=1  v_capacitor_nominal_unit=V  Qj_specify=off  Qj_priority=High  Qj=0 C  Qj_nominal_specify=off  Qj_nominal_value=1  Qj_nominal_unit=C  i_diode_specify=off  i_diode_priority=None  i_diode=0 A  i_diode_nominal_specify=off  i_diode_nominal_value=1  i_diode_nominal_unit=A  v_diode_specify=off  v_diode_priority=None  v_diode=0 V  v_diode_nominal_specify=off  v_diode_nominal_value=1  v_diode_nominal_unit=V  i_capacitor_specify=off  i_capacitor_priority=None  i_capacitor=0 A  i_capacitor_nominal_specify=off  i_capacitor_nominal_value=1  i_capacitor_nominal_unit=A  power_dissipated_specify=off  power_dissipated_priority=None  power_dissipated=0 W  power_dissipated_nominal_specify=off  power_dissipated_nominal_value=1  power_dissipated_nominal_unit=W  fidelity_level=ee.enum.diode.fidelity.includeChargeDyn  rec_loss_model=ee.enum.diode.reverseRecoveryModel.fixed  ErecVal=0 J  scaleWithIandV=true  ErecMat=zeros(2, 3) J  TjrecVec=[298.15, 398.15] K  IfrecVec=[.1, 1, 10] A  IrecVal=10 A  VrecVal=10 V  tFilter=1 / 1000 / 100 s  thermal_network_parameterization=ee.enum.thermalNetworkTopology.junctionCase  Rth=[0, 10] K/W  Rth_Cauer=[1, 3, 10] K/W  Rth_Foster=[.08, .14, .22, .16] K/W  thermal_mass_parameterization=ee.enum.thermalNetwork.timeconstant  thermal_mass=[0, 1] J/K  thermal_mass_Cauer=[.1, .3, 1] J/K  thermal_mass_Foster=[.001, .005, .05, .5] J/K  thermal_time_constant=[0, 10] s  thermal_time_constant_Cauer=[1, 3, 10] s  thermal_time_constant_Foster=[7e-05, .0007, .01, .08] s  thermal_mass_initial_temperatures=[25, 25] degC  thermal_mass_initial_temperatures_Cauer=[25, 25, 25] degC  junction_thermal_mass=0.01 J/K  Tvec_initial_Foster=[25, 25, 25, 25] degC  no_thermal_network=0  junction_temperature_specify=off  junction_temperature_priority=None  junction_temperature=25 degC  junction_temperature_nominal_specify=off  junction_temperature_nominal_value=1  junction_temperature_nominal_unit=degC
  LPF Voltage: 2nd Order 20kHz : TransferFcn  Numerator=[(2*pi*20000)^2]  Denominator=[1, sqrt(2)*(2*pi*20000), (2*pi*20000)^2]
  PS-Simulink Converter : nesl_utility/PS-Simulink Converter  PhysicalDomain=network_engine_domain  SubClassName=ps_output  LeftPortType=input  RightPortType=output  PseudoPeriodic=off  Frequencies=[]  VectorFormat=inherit  Unit=inherit  AffineConversion=off
  PS-Simulink Converter1 : nesl_utility/PS-Simulink Converter  PhysicalDomain=network_engine_domain  SubClassName=ps_output  LeftPortType=input  RightPortType=output  PseudoPeriodic=off  Frequencies=[]  VectorFormat=inherit  Unit=inherit  AffineConversion=off
  Simulink-PS Converter : nesl_utility/Simulink-PS Converter  PhysicalDomain=network_engine_domain  SubClassName=ps_input  LeftPortType=input  RightPortType=output  PseudoPeriodic=off  Frequencies=[]  NoiseDistribution=none  NoiseParameters=[]  Unit=1  AffineConversion=off  FilteringAndDerivatives=provide  SimscapeFilterOrder=1  InputFilterTimeConstant=0.001  UdotUserProvided=0
  Solar Cell : ee_lib/Sources/Solar Cell  prm=ee.enum.sources.solar_cell_prm.fiveParameter  Isc=7.34 A  Voc=0.6 V  Is=1.728e-12 A  Is2=0 A  Iph=14.96 A  Ir0=1000 W/m^2  ec=1  N2=2  Rs=0.00263 Ohm  Rp=inf Ohm  N_series=60  N_parallel=1  TIPH1=0.0005 1/K  EG=1.11 eV  TXIS1=3  TXIS2=3  TRS1=0  TRP1=0  Tmeas=25 degC  TFIXED=25 degC  thermal_mass=100 J/K  initial_temperature=25 degC
  Voltage Sensor : fl_lib/Electrical/Electrical Sensors/Voltage Sensor
  +ve Terminal : PMIOPort  Side=Left
  -ve Terminal : PMIOPort  Port=2  Side=Left
  VM4 : Outport
  IM4 : Outport  Port=2
  wires:
  In_Irrad/1 -> Simulink-PS Converter/1
  PS-Simulink Converter1/1 -> LPF Voltage: 2nd Order 20kHz/1
  PS-Simulink Converter/1 -> IM4/1
  LPF Voltage: 2nd Order 20kHz/1 -> VM4/1
  connections:
  -ve Terminal/RConn1 -- Diode/LConn1 -- Voltage Sensor/RConn2 -- Solar Cell/RConn1
  Solar Cell/LConn2 -- Diode/RConn1 -- Current Sensor/LConn1
  Simulink-PS Converter/RConn1 -- Solar Cell/LConn1
  Current Sensor/RConn2 -- Voltage Sensor/LConn1 -- +ve Terminal/RConn1
  Voltage Sensor/RConn1 -- PS-Simulink Converter1/LConn1
  PS-Simulink Converter/LConn1 -- Current Sensor/RConn1
